simulink model "mult_test2"  (Simulink 5.0)
settings: Solver=ode45  StartTime=0.0  StopTime=10.0  RelTol=1e-3
values from neighbouring files (symbols this model uses):
  P0 = covupdate(P1,K,H)    [casimple.m]    (also in cmigits28_model_01.mat = [100 0 0 0 0 0 0 0 0 0 0 0 ... (784 elements, 28x28)])
settings Model: Creator=mcarroll  LastModifiedBy=mcarroll  ExtModeAutoUpdateStatusClock=off

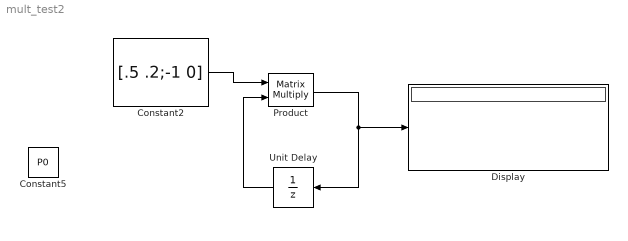
== system mult_test2 ==
  Constant2 : Constant  Value=[.5 .2;-1 0]  VectorParams1D=off
  Constant5 : Constant  Value=P0  VectorParams1D=off
  Display : Display
  Product : Product  Multiplication=Matrix(*)  SaturateOnIntegerOverflow=on
  Unit Delay : UnitDelay  Orientation=left  X0=P0
  wires:
  Constant2/1 -> Product/1
  Product/1 -> Display/1, Unit Delay/1
  Unit Delay/1 -> Product/2
